simulink model "ex2s"  (R2022a)
settings: Solver=VariableStepAuto  StartTime=0.0  StopTime=10.0  RelTol=1e-3
libraries: nesl_utility x2
settings Model: Creator=giova  LastModifiedBy=giova

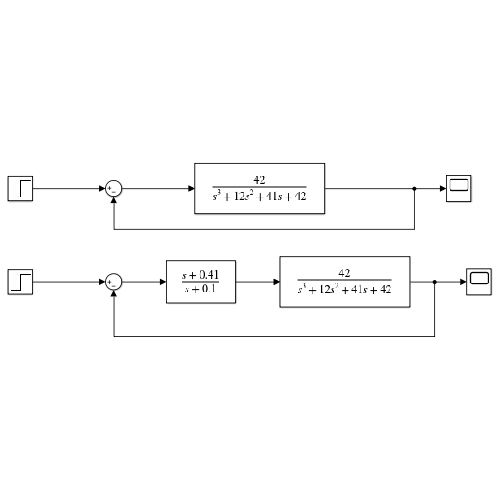
[thumbnail: Simulink's stored preview of the top-level diagram]
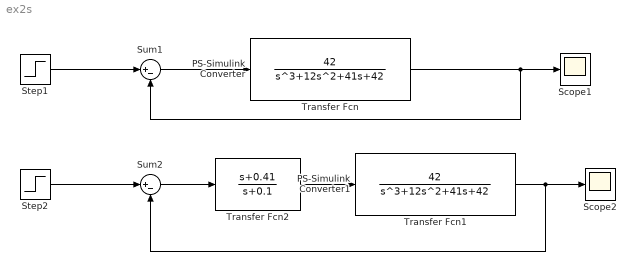
== system ex2s ==
  PS-Simulink Converter : nesl_utility/PS-Simulink Converter  PhysicalDomain=network_engine_domain  SubClassName=ps_output  LeftPortType=input  RightPortType=output  PseudoPeriodic=off  Frequencies=[]  VectorFormat=inherit  Unit=inherit  AffineConversion=off
      settings: SourceProductBaseCode=SS,PW,VE
  PS-Simulink Converter1 : nesl_utility/PS-Simulink Converter  PhysicalDomain=network_engine_domain  SubClassName=ps_output  LeftPortType=input  RightPortType=output  PseudoPeriodic=off  Frequencies=[]  VectorFormat=inherit  Unit=inherit  AffineConversion=off
      settings: SourceProductBaseCode=SS,PW,VE
  Scope1 : Scope
  Scope2 : Scope
  Step1 : Step  SampleTime=0
  Step2 : Step  SampleTime=0
  Sum1 : Sum  Inputs=|+-
  Sum2 : Sum  Inputs=|+-
  Transfer Fcn : TransferFcn  Numerator=[42]  Denominator=[1 12 41 42]
  Transfer Fcn1 : TransferFcn  Numerator=[42]  Denominator=[1 12 41 42]
  Transfer Fcn2 : TransferFcn  Numerator=[1 0.41]  Denominator=[1 0.1]
  wires:
  Step1/1 -> Sum1/1
  Transfer Fcn/1 -> Sum1/2, Scope1/1
  Sum1/1 -> Transfer Fcn/1
  Transfer Fcn1/1 -> Sum2/2, Scope2/1
  Step2/1 -> Sum2/1
  Sum2/1 -> Transfer Fcn2/1
  Transfer Fcn2/1 -> Transfer Fcn1/1
